simulink model "EMG_Gripper_System"  (R2025a)
settings: Solver=FixedStepDiscrete  StartTime=0  StopTime=10  FixedStep=0.005  RelTol=1e-3
undefined symbols (not defined in the file): dspblkCoreblockFVToolHelper, gcbh
settings Model: Creator=mahdi  LastModifiedBy=mahdi

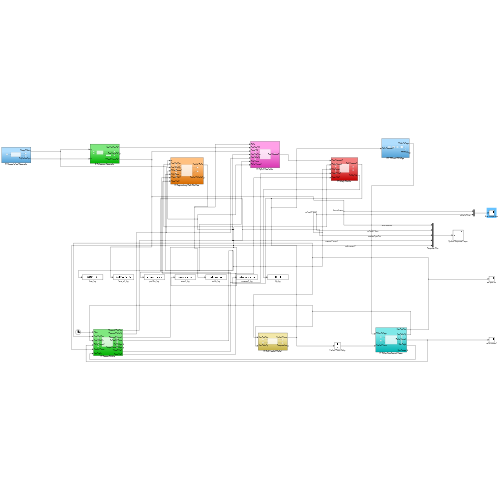
[thumbnail: Simulink's stored preview of the top-level diagram]
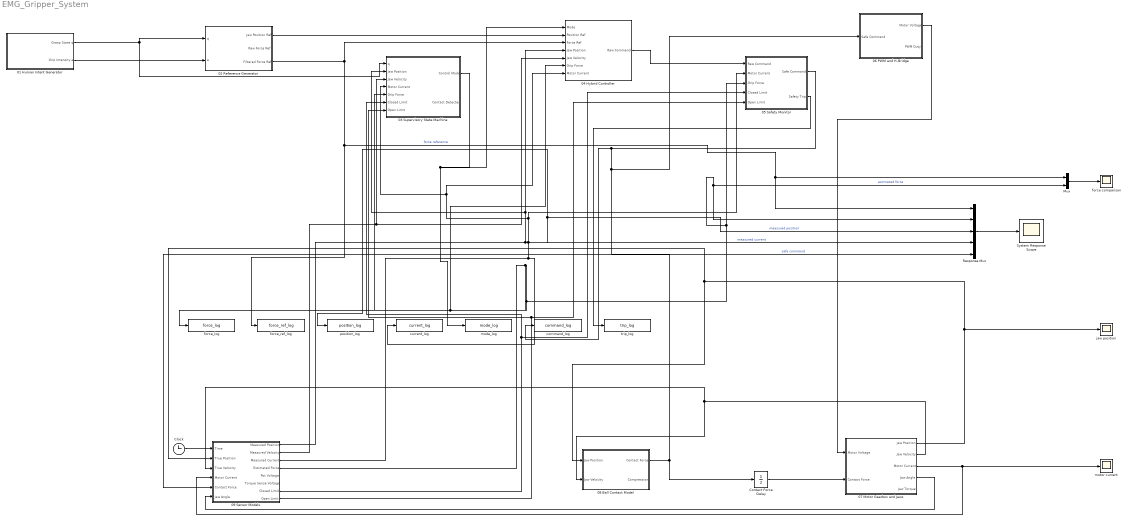
== system EMG_Gripper_System ==
  01 Human Intent Generator : Subsystem
  02 Reference Generator : Subsystem
  03 Supervisory State Machine : Subsystem
  04 Hybrid Controller : Subsystem
  05 Safety Monitor : Subsystem
  06 PWM and H-Bridge : Subsystem
  07 Motor Gearbox and Jaws : Subsystem
  08 Ball Contact Model : Subsystem
  09 Sensor Models : Subsystem
  Clock : Clock
  Contact Force Delay : UnitDelay  SampleTime=0.005  HasFrameUpgradeWarning=on
  Mux : Mux  Inputs=2
  Response Mux : Mux  Inputs=5
  System Response Scope : Scope
      settings: ActiveDisplayYMinimum=-1  ActiveDisplayYMaximum=1
  command_log : ToWorkspace  VariableName=command_log  SaveFormat=Timeseries  SampleTime=-1
  current_log : ToWorkspace  VariableName=current_log  SaveFormat=Timeseries  SampleTime=-1
  force comparison : Scope
      settings: ActiveDisplayYMinimum=-1.0387902929398534  ActiveDisplayYMaximum=16.21858095876355
  force_log : ToWorkspace  VariableName=force_log  SaveFormat=Timeseries  SampleTime=-1
  force_ref_log : ToWorkspace  VariableName=force_ref_log  SaveFormat=Timeseries  SampleTime=-1
  jaw position : Scope
      settings: ActiveDisplayYMinimum=-1  ActiveDisplayYMaximum=1  DataLoggingVariableName=ScopeData2
  mode_log : ToWorkspace  VariableName=mode_log  SaveFormat=Timeseries  SampleTime=-1
  motor current : Scope
      settings: ActiveDisplayYMinimum=-1  ActiveDisplayYMaximum=1  DataLoggingVariableName=ScopeData3
  position_log : ToWorkspace  VariableName=position_log  SaveFormat=Timeseries  SampleTime=-1
  trip_log : ToWorkspace  VariableName=trip_log  SaveFormat=Timeseries  SampleTime=-1
  wires:
  01 Human Intent Generator/1(Grasp State q) -> 02 Reference Generator/1(q), 03 Supervisory State Machine/1(q)
  01 Human Intent Generator/2(Grip Intensity a) -> 02 Reference Generator/2(a)
  02 Reference Generator/1(Jaw Position Ref) -> 04 Hybrid Controller/2(Position Ref)
  02 Reference Generator/3(Filtered Force Ref) -> 04 Hybrid Controller/3(Force Ref), force_ref_log/1, Response Mux/1, Mux/1  "force reference"
  03 Supervisory State Machine/1(Control Mode) -> 04 Hybrid Controller/1(Mode), mode_log/1
  04 Hybrid Controller/1(Raw Command) -> 05 Safety Monitor/1(Raw Command)
  05 Safety Monitor/1(Safe Command) -> 06 PWM and H-Bridge/1(Safe Command), Response Mux/5, command_log/1  "safe command"
  06 PWM and H-Bridge/1(Motor Voltage) -> 07 Motor Gearbox and Jaws/1(Motor Voltage)
  07 Motor Gearbox and Jaws/2(Jaw Velocity) -> 09 Sensor Models/3(True Velocity), 08 Ball Contact Model/2(Jaw Velocity)
  08 Ball Contact Model/1(Contact Force) -> 09 Sensor Models/5(Contact Force), Contact Force Delay/1
  Contact Force Delay/1 -> 07 Motor Gearbox and Jaws/2(Contact Force)
  Clock/1 -> 09 Sensor Models/1(Time)
  07 Motor Gearbox and Jaws/3(Motor Current) -> motor current/1, 09 Sensor Models/4(Motor Current)
  07 Motor Gearbox and Jaws/4(Jaw Angle) -> 09 Sensor Models/6(Jaw Angle)
  09 Sensor Models/1(Measured Position) -> Response Mux/3, position_log/1, 03 Supervisory State Machine/2(Jaw Position), 04 Hybrid Controller/4(Jaw Position)  "measured position"
  09 Sensor Models/2(Measured Velocity) -> 04 Hybrid Controller/5(Jaw Velocity), 03 Supervisory State Machine/3(Jaw Velocity)
  09 Sensor Models/3(Measured Current) -> 05 Safety Monitor/2(Motor Current), 03 Supervisory State Machine/4(Motor Current), 04 Hybrid Controller/7(Motor Current), Response Mux/4, current_log/1  "measured current"
  09 Sensor Models/4(Estimated Force) -> Response Mux/2, Mux/2, 05 Safety Monitor/3(Grip Force), force_log/1, 04 Hybrid Controller/6(Grip Force), 03 Supervisory State Machine/5(Grip Force)  "estimated force"
  09 Sensor Models/7(Closed Limit) -> 03 Supervisory State Machine/6(Closed Limit), 05 Safety Monitor/4(Closed Limit)
  09 Sensor Models/8(Open Limit) -> 05 Safety Monitor/5(Open Limit), 03 Supervisory State Machine/7(Open Limit)
  05 Safety Monitor/2(Safety Trip) -> trip_log/1
  Response Mux/1 -> System Response Scope/1
  Mux/1 -> force comparison/1
  07 Motor Gearbox and Jaws/1(Jaw Position) -> 09 Sensor Models/2(True Position), 08 Ball Contact Model/1(Jaw Position), jaw position/1

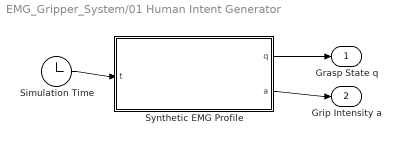
== system EMG_Gripper_System/01 Human Intent Generator ==
  Simulation Time : Clock
  Synthetic EMG Profile : MATLAB Function  TreatAsAtomicUnit=on
  Grasp State q : Outport
  Grip Intensity a : Outport  Port=2
  wires:
  Simulation Time/1 -> Synthetic EMG Profile/1(t)
  Synthetic EMG Profile/1(q) -> Grasp State q/1
  Synthetic EMG Profile/2(a) -> Grip Intensity a/1

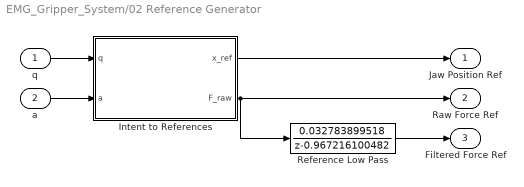
== system EMG_Gripper_System/02 Reference Generator ==
  q : Inport
  a : Inport  Port=2
  Intent to References : MATLAB Function  TreatAsAtomicUnit=on
  Reference Low Pass : DiscreteTransferFcn  LoadFcn=dspblkCoreblockFVToolHelper(gcbh,'load');  Numerator=0.032783899518  Denominator=[1 -0.967216100482]  SampleTime=0.005
      settings: CopyFcn=dspblkCoreblockFVToolHelper(gcbh,'copy');  DeleteFcn=dspblkCoreblockFVToolHelper(gcbh,'close');  ModelCloseFcn=dspblkCoreblockFVToolHelper(gcbh,'close');  PreSaveFcn=dspblkCoreblockFVToolHelper(gcbh,'presave');  PostSaveFcn=dspblkCoreblockFVToolHelper(gcbh,'postsave');  CloseFcn=dspblkCoreblockFVToolHelper(gcbh,'close');
  Jaw Position Ref : Outport
  Raw Force Ref : Outport  Port=2
  Filtered Force Ref : Outport  Port=3
  wires:
  q/1 -> Intent to References/1(q)
  a/1 -> Intent to References/2(a)
  Intent to References/1(x_ref) -> Jaw Position Ref/1
  Intent to References/2(F_raw) -> Raw Force Ref/1, Reference Low Pass/1
  Reference Low Pass/1 -> Filtered Force Ref/1

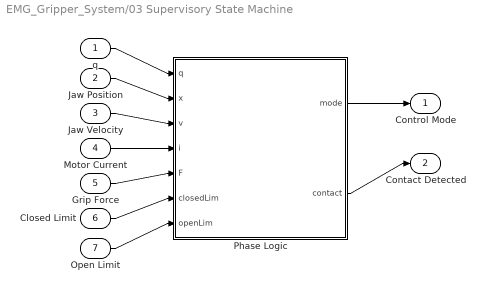
== system EMG_Gripper_System/03 Supervisory State Machine ==
  q : Inport
  Jaw Position : Inport  Port=2
  Jaw Velocity : Inport  Port=3
  Motor Current : Inport  Port=4
  Grip Force : Inport  Port=5
  Closed Limit : Inport  Port=6
  Open Limit : Inport  Port=7
  Phase Logic : MATLAB Function  TreatAsAtomicUnit=on
  Control Mode : Outport
  Contact Detected : Outport  Port=2
  wires:
  q/1 -> Phase Logic/1(q)
  Jaw Position/1 -> Phase Logic/2(x)
  Jaw Velocity/1 -> Phase Logic/3(v)
  Motor Current/1 -> Phase Logic/4(i)
  Grip Force/1 -> Phase Logic/5(F)
  Closed Limit/1 -> Phase Logic/6(closedLim)
  Open Limit/1 -> Phase Logic/7(openLim)
  Phase Logic/1(mode) -> Control Mode/1
  Phase Logic/2(contact) -> Contact Detected/1

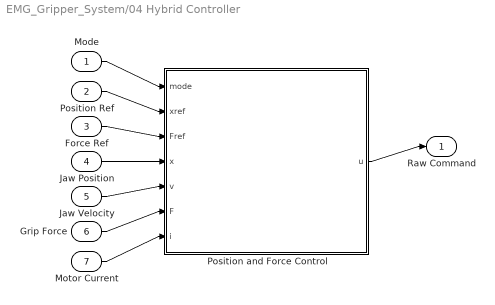
== system EMG_Gripper_System/04 Hybrid Controller ==
  Mode : Inport
  Position Ref : Inport  Port=2
  Force Ref : Inport  Port=3
  Jaw Position : Inport  Port=4
  Jaw Velocity : Inport  Port=5
  Grip Force : Inport  Port=6
  Motor Current : Inport  Port=7
  Position and Force Control : MATLAB Function  TreatAsAtomicUnit=on
  Raw Command : Outport
  wires:
  Mode/1 -> Position and Force Control/1(mode)
  Position Ref/1 -> Position and Force Control/2(xref)
  Force Ref/1 -> Position and Force Control/3(Fref)
  Jaw Position/1 -> Position and Force Control/4(x)
  Jaw Velocity/1 -> Position and Force Control/5(v)
  Grip Force/1 -> Position and Force Control/6(F)
  Motor Current/1 -> Position and Force Control/7(i)
  Position and Force Control/1(u) -> Raw Command/1

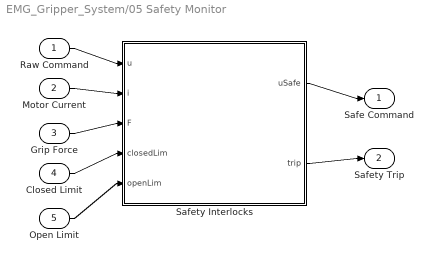
== system EMG_Gripper_System/05 Safety Monitor ==
  Raw Command : Inport
  Motor Current : Inport  Port=2
  Grip Force : Inport  Port=3
  Closed Limit : Inport  Port=4
  Open Limit : Inport  Port=5
  Safety Interlocks : MATLAB Function  TreatAsAtomicUnit=on
  Safe Command : Outport
  Safety Trip : Outport  Port=2
  wires:
  Raw Command/1 -> Safety Interlocks/1(u)
  Motor Current/1 -> Safety Interlocks/2(i)
  Grip Force/1 -> Safety Interlocks/3(F)
  Closed Limit/1 -> Safety Interlocks/4(closedLim)
  Open Limit/1 -> Safety Interlocks/5(openLim)
  Safety Interlocks/1(uSafe) -> Safe Command/1
  Safety Interlocks/2(trip) -> Safety Trip/1

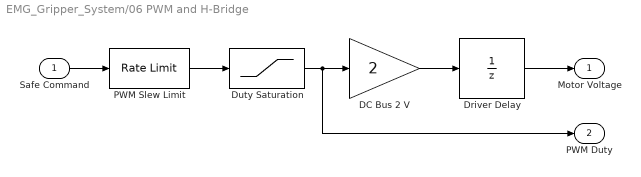
== system EMG_Gripper_System/06 PWM and H-Bridge ==
  Safe Command : Inport
  DC Bus 2 V : Gain  Gain=2
  Driver Delay : UnitDelay  SampleTime=0.005  HasFrameUpgradeWarning=on
  Duty Saturation : Saturate  UpperLimit=1  LowerLimit=-1
  PWM Slew Limit : RateLimiter  RisingSlewLimit=6  FallingSlewLimit=-6  SampleTimeMode=inherited
  Motor Voltage : Outport
  PWM Duty : Outport  Port=2
  wires:
  Safe Command/1 -> PWM Slew Limit/1
  PWM Slew Limit/1 -> Duty Saturation/1
  Duty Saturation/1 -> DC Bus 2 V/1, PWM Duty/1
  DC Bus 2 V/1 -> Driver Delay/1
  Driver Delay/1 -> Motor Voltage/1

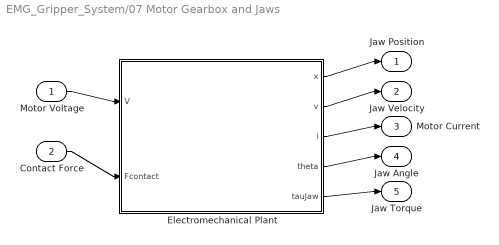
== system EMG_Gripper_System/07 Motor Gearbox and Jaws ==
  Motor Voltage : Inport
  Contact Force : Inport  Port=2
  Electromechanical Plant : MATLAB Function  TreatAsAtomicUnit=on
  Jaw Position : Outport
  Jaw Velocity : Outport  Port=2
  Motor Current : Outport  Port=3
  Jaw Angle : Outport  Port=4
  Jaw Torque : Outport  Port=5
  wires:
  Motor Voltage/1 -> Electromechanical Plant/1(V)
  Contact Force/1 -> Electromechanical Plant/2(Fcontact)
  Electromechanical Plant/1(x) -> Jaw Position/1
  Electromechanical Plant/2(v) -> Jaw Velocity/1
  Electromechanical Plant/3(i) -> Motor Current/1
  Electromechanical Plant/4(theta) -> Jaw Angle/1
  Electromechanical Plant/5(tauJaw) -> Jaw Torque/1

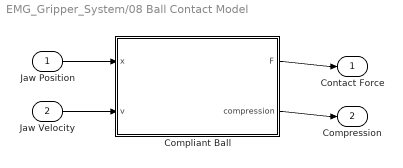
== system EMG_Gripper_System/08 Ball Contact Model ==
  Jaw Position : Inport
  Jaw Velocity : Inport  Port=2
  Compliant Ball : MATLAB Function  TreatAsAtomicUnit=on
  Contact Force : Outport
  Compression : Outport  Port=2
  wires:
  Jaw Position/1 -> Compliant Ball/1(x)
  Jaw Velocity/1 -> Compliant Ball/2(v)
  Compliant Ball/1(F) -> Contact Force/1
  Compliant Ball/2(compression) -> Compression/1

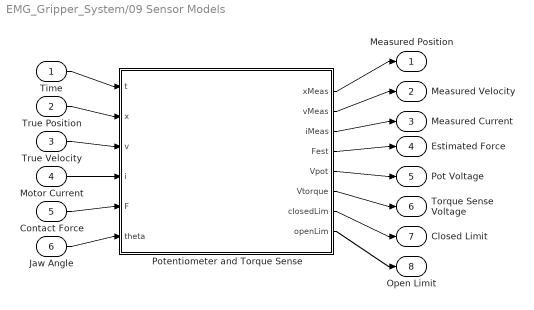
== system EMG_Gripper_System/09 Sensor Models ==
  Time : Inport
  True Position : Inport  Port=2
  True Velocity : Inport  Port=3
  Motor Current : Inport  Port=4
  Contact Force : Inport  Port=5
  Jaw Angle : Inport  Port=6
  Potentiometer and Torque Sense : MATLAB Function  TreatAsAtomicUnit=on
  Measured Position : Outport
  Measured Velocity : Outport  Port=2
  Measured Current : Outport  Port=3
  Estimated Force : Outport  Port=4
  Pot Voltage : Outport  Port=5
  Torque Sense Voltage : Outport  Port=6
  Closed Limit : Outport  Port=7
  Open Limit : Outport  Port=8
  wires:
  Time/1 -> Potentiometer and Torque Sense/1(t)
  True Position/1 -> Potentiometer and Torque Sense/2(x)
  True Velocity/1 -> Potentiometer and Torque Sense/3(v)
  Motor Current/1 -> Potentiometer and Torque Sense/4(i)
  Contact Force/1 -> Potentiometer and Torque Sense/5(F)
  Jaw Angle/1 -> Potentiometer and Torque Sense/6(theta)
  Potentiometer and Torque Sense/1(xMeas) -> Measured Position/1
  Potentiometer and Torque Sense/2(vMeas) -> Measured Velocity/1
  Potentiometer and Torque Sense/3(iMeas) -> Measured Current/1
  Potentiometer and Torque Sense/4(Fest) -> Estimated Force/1
  Potentiometer and Torque Sense/5(Vpot) -> Pot Voltage/1
  Potentiometer and Torque Sense/6(Vtorque) -> Torque Sense Voltage/1
  Potentiometer and Torque Sense/7(closedLim) -> Closed Limit/1
  Potentiometer and Torque Sense/8(openLim) -> Open Limit/1

== matlab function EMG_Gripper_System/02 Reference Generator/Intent to References ==
  data: q input; x_ref output; a input; F_raw output
function [x_ref,F_raw] = fcn(q,a)
% Opening range is 0 to 2 inches; safe force command is 5 to 18 N.
x_max = 0.0508;
a = min(max(a,0),1);
if q == 0 || q == 3
    x_ref = x_max; F_raw = 0;
else
    x_ref = 0; F_raw = 5 + 13*a;
end

== matlab function EMG_Gripper_System/01 Human Intent Generator/Synthetic EMG Profile ==
  data: t input; q output; a output
function [q,a] = fcn(t)
% q: 0 OPEN, 1 GRIPPING, 2 HOLDING, 3 RELEASING
if t < 1
    q = 0; a = 0;
elseif t < 2
    q = 1; a = 0.5*(t-1);
elseif t < 5
    q = 2; a = 0.5;
elseif t < 6
    q = 2; a = 0.5 + 0.3*(t-5);
% elseif t < 7
%     q = 2; a = 0.5 + 0.1*(t-6);
elseif t < 8
    q = 2; a = 0.8;
elseif t < 9
    q = 3; a = 0.8*(9-t);
else
    q = 0; a = 0;
end

== matlab function EMG_Gripper_System/03 Supervisory State Machine/Phase Logic ==
  data: q input; mode output; x input; v input; i input; F input; closedLim input; openLim input; contact output
function [mode,contact] = fcn(q,x,v,i,F,closedLim,openLim)
% mode: 0 OPEN, 1 APPROACH, 2 FORCE, 3 HOLD, 4 RELEASE
contact = double((F > 1.0) || ((abs(i) > 0.08) && (abs(v) < 0.0025)));
if q == 0
    mode = 0;
elseif q == 3
    mode = 4;
elseif q == 1
    if contact || closedLim
        mode = 2;
    else
        mode = 1;
    end
else
    mode = 3;
end
if openLim && q == 0
    mode = 0;
end

== matlab function EMG_Gripper_System/04 Hybrid Controller/Position and Force Control ==
  data: mode input; u output; xref input; Fref input; x input; v input; F input; i input
function u = fcn(mode,xref,Fref,x,v,F,i)
% Discrete hybrid controller, Ts = 5 ms. Positive command opens jaws.
persistent iF prevMode
if isempty(iF), iF = 0; prevMode = -1; end
Ts = 0.005;
if mode ~= prevMode, iF = 0; end
if mode == 0 || mode == 4
    % Position PD for OPEN and RELEASE.
    u = 28*(xref-x) - 1.5*v;
elseif mode == 1
    % Controlled approach velocity.
    u = -0.55 - 6*x;
else
    % PI force control in GRIP/HOLD. Closing command is negative.
    e = Fref-F;
    iCandidate = min(max(iF + Ts*e,-30),30);
    uUnsat = -(0.018*e + 0.10*iCandidate);
    u = min(max(uUnsat,-1),1);
    if abs(uUnsat) < 1, iF = iCandidate; end
end
u = min(max(u,-1),1);
prevMode = mode;

== matlab function EMG_Gripper_System/05 Safety Monitor/Safety Interlocks ==
  data: u input; uSafe output; i input; F input; closedLim input; openLim input; trip output
function [uSafe,trip] = fcn(u,i,F,closedLim,openLim)
% 70% of the 2 V stall current and 70% of 178 N datasheet peak.
Imax = 0.70*(2/8.5);
Fmax = 0.70*178;
% A 0.7 duty cap on the 2 V bus guarantees <=70% stall current.
uSafe = min(max(u,-0.7),0.7); trip = 0;
if ((abs(i) > 1.02*Imax) && (sign(uSafe)==sign(i))) || (F >= Fmax && uSafe < 0)
    uSafe = 0; trip = 1;
end
if closedLim && uSafe < -0.02, uSafe = 0; trip = 1; end
if openLim && uSafe > 0.02, uSafe = 0; trip = 1; end
if ~isfinite(uSafe), uSafe = 0; trip = 1; end

== matlab function EMG_Gripper_System/07 Motor Gearbox and Jaws/Electromechanical Plant ==
  data: V input; x output; Fcontact input; v output; i output; theta output; tauJaw output
function [x,v,i,theta,tauJaw] = fcn(V,Fcontact)
% Discrete nonlinear gripper plant. Outputs are pre-update states.
persistent th w
if isempty(th), th = pi/2; w = 0; end
Ts=0.005; R=8.5; Kt=0.31*0.00706155; Ke=Kt;
Ng=49.3; Nj=50; eta=0.50; J=0.12; B=0.40;
r=0.03175; xMax=0.0508;
x = xMax*th/(pi/2); v = xMax*w/(pi/2); theta = th;
i = min(max((V-Ke*Ng*w)/R,-0.5),0.5);
tauJaw = eta*Ng*Nj*Kt*i;
thetaEff=max(th,7*pi/180);
tauContact = max(Fcontact,0)*r*sin(thetaEff);
tauNet = tauJaw + tauContact - B*w;
wNew = w + Ts*tauNet/J;
thNew = th + Ts*wNew;
if thNew <= 0, thNew=0; wNew=max(wNew,0); end
if thNew >= pi/2, thNew=pi/2; wNew=min(wNew,0); end
th=thNew; w=wNew;

== matlab function EMG_Gripper_System/08 Ball Contact Model/Compliant Ball ==
  data: x input; F output; v input; compression output
function [F,compression] = fcn(x,v)
% 32 mm object, Kelvin-Voigt contact, force capped at safe peak.
diameter=0.032; k=4500; c=35;
compression=max(diameter-x,0);
if compression > 0
    F=max(k*compression+c*max(-v,0),0);
else
    F=0;
end
F=min(F,124.6);

== matlab function EMG_Gripper_System/09 Sensor Models/Potentiometer and Torque Sense ==
  data: t input; xMeas output; x input; v input; i input; F input; theta input; vMeas output; iMeas output; Fest output; Vpot output; Vtorque output; closedLim output; openLim output
function [xMeas,vMeas,iMeas,Fest,Vpot,Vtorque,closedLim,openLim] = fcn(t,x,v,i,F,theta)
% Datasheet sensor relations with deterministic low-level ripple.
Vexc=5; Rtorque=1; Kt=0.31*0.00706155; Ng=49.3; Nj=50; eta=0.50; r=0.03175;
xMeas=min(max(x + 2e-5*sin(2*pi*17*t),0),0.0508);
vMeas=v; iMeas=i + 5e-4*sin(2*pi*23*t);
Vpot=(Vexc/3)*(theta/(pi/2));
Vtorque=abs(iMeas)*Rtorque;
thetaEff=max(theta,7*pi/180);
if F >= 0.5 && iMeas < 0    
    Fest = max(-eta*Ng*Nj*Kt*iMeas ...
        /(r*sin(thetaEff)), 0);
else
    Fest = 0;
end
if F < 0.5, Fest=0; end
closedLim = double(x <= 2e-4); openLim = double(x >= (0.0508-2e-4));
